simulink model "s_c_nbe_m32k"  (R2018a)
settings: Solver=VariableStepDiscrete  StartTime=0.0  StopTime=1000  RelTol=1e-3
undefined symbols (not defined in the file): fft_stages, n_taps, output_bits, pfb_coeff_gen_calc, xengbits
libraries: xbsIndex_r4 x23714, casper_library_misc x17, xps_library x4, casper_library_scopes x4, xbsReplacements_r4 x4
(part 45 of 171)

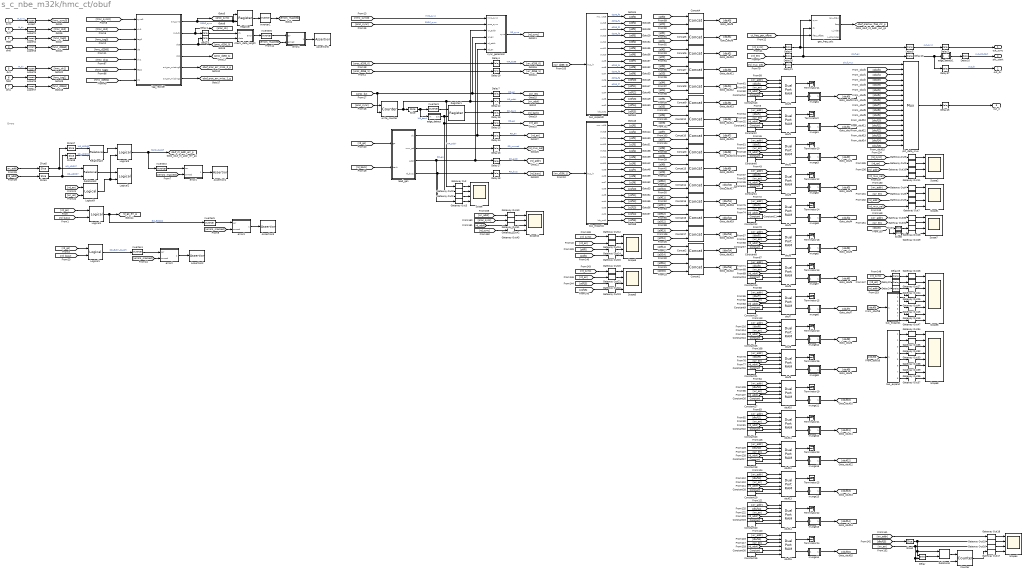
== system s_c_nbe_m32k/hmc_ct/obuf ==
  note: Errors
  sync : Inport
  dv0 : Inport  Port=2
  tag0 : Inport  Port=3
  din0 : Inport  Port=4
  dv1 : Inport  Port=5
  tag1 : Inport  Port=6
  din1 : Inport  Port=7
  Assert : xbsIndex_r4/Assert  assert_type=on  type_source=Explicitly  gui_display_data_type=Boolean  arith_type=Boolean  n_bits=16  bin_pt=14  preci_type=Single  exp_width=8  frac_width=24  assert_rate=on  rate_source=Explicitly  period=1  output_port=on  block_type=assert
  Assert1 : xbsIndex_r4/Assert  assert_type=on  type_source=Explicitly  gui_display_data_type=Boolean  arith_type=Boolean  n_bits=16  bin_pt=14  preci_type=Single  exp_width=8  frac_width=24  assert_rate=on  rate_source=Explicitly  period=1  output_port=on  block_type=assert
  Assert2 : xbsIndex_r4/Assert  assert_type=on  type_source=Explicitly  gui_display_data_type=Fixed-point  arith_type=Unsigned  n_bits=9  bin_pt=0  preci_type=Single  exp_width=8  frac_width=24  assert_rate=on  rate_source=Explicitly  period=1  output_port=on  block_type=assert
  Assert3 : xbsIndex_r4/Assert  assert_type=on  type_source=Explicitly  gui_display_data_type=Fixed-point  arith_type=Unsigned  n_bits=256  bin_pt=0  preci_type=Single  exp_width=8  frac_width=24  assert_rate=on  rate_source=Explicitly  period=1  output_port=on  block_type=assert
  Assert5 : xbsIndex_r4/Assert  assert_type=on  type_source=Explicitly  gui_display_data_type=Boolean  arith_type=Boolean  n_bits=16  bin_pt=14  preci_type=Single  exp_width=8  frac_width=24  assert_rate=on  rate_source=Explicitly  period=1  output_port=on  block_type=assert
  Assert6 : xbsIndex_r4/Assert  assert_type=on  type_source=Explicitly  gui_display_data_type=Fixed-point  arith_type=Unsigned  n_bits=9  bin_pt=0  preci_type=Single  exp_width=8  frac_width=24  assert_rate=on  rate_source=Explicitly  period=1  output_port=on  block_type=assert
  Assert7 : xbsIndex_r4/Assert  assert_type=on  type_source=Explicitly  gui_display_data_type=Fixed-point  arith_type=Unsigned  n_bits=256  bin_pt=0  preci_type=Single  exp_width=8  frac_width=24  assert_rate=on  rate_source=Explicitly  period=1  output_port=on  block_type=assert
  Assertion{1..3,5} (4 alike) : Assertion  Enabled=off
  Concat{1..10,12..17} (16 alike) : xbsIndex_r4/Concat  num_inputs=2  dbl_ovrd=off  block_type=concat
  Constant{1,3,5,7,9,11,13,15,17,19,22,24,26,28,30,42} (16 alike) : xbsIndex_r4/Constant  const=0  gui_display_data_type=Fixed-point  arith_type=Unsigned  n_bits=256  bin_pt=0  preci_type=Single  exp_width=8  frac_width=24  explicit_period=on  period=1  equ=P=C  opselect=C  inp2=PCIN>>17  opr=+  inp1=P  carry=CIN  dbl_ovrd=off  block_type=constant
  Constant{2,4,6,8,10,12,14,16,18,20..21,23,25,27,29,43} (16 alike) : xbsIndex_r4/Constant  const=0  gui_display_data_type=Boolean  arith_type=Boolean  n_bits=256  bin_pt=0  preci_type=Single  exp_width=8  frac_width=24  explicit_period=on  period=1  equ=P=C  opselect=C  inp2=PCIN>>17  opr=+  inp1=P  carry=CIN  dbl_ovrd=off  block_type=constant
  Counter : xbsIndex_r4/Counter  cnt_type=Free Running  cnt_to=Inf  operation=Up  start_count=0  cnt_by_val=1  arith_type=Unsigned  n_bits=8  bin_pt=0  load_pin=off  rst=on  en=on  explicit_period=on  period=1  use_behavioral_HDL=off  implementation=Fabric  dbl_ovrd=off  block_type=counter
  Delay : xbsIndex_r4/Delay  rst=off  infoeditControl=Selection of Reset will increase slice count due to use of real FFs and instead of SRLs  en=on  latency=1  reg_retiming=off  dbl_ovrd=off  block_type=delay
      settings: infoedit=Hardware notes: A delay line is a chain, each link of which is an SRL16 or SRL32 followed by a flip-flop.
  Delay1 : xbsIndex_r4/Delay  rst=off  infoeditControl=Selection of Reset will increase slice count due to use of real FFs and instead of SRLs  en=off  latency=1  reg_retiming=on  dbl_ovrd=off  block_type=delay
      settings: infoedit=Hardware notes: A delay line is a chain, each link of which is an SRL16 or SRL32 followed by a flip-flop.
  Delay{4,7,10,12..19} (11 alike) : xbsIndex_r4/Delay  rst=off  infoeditControl=Selection of Reset will increase slice count due to use of real FFs and instead of SRLs  en=off  latency=2  reg_retiming=on  dbl_ovrd=off  block_type=delay
      settings: infoedit=Hardware notes: A delay line is a chain, each link of which is an SRL16 or SRL32 followed by a flip-flop.
  Delay2 : xbsIndex_r4/Delay  rst=off  infoeditControl=Selection of Reset will increase slice count due to use of real FFs and instead of SRLs  en=off  latency=1  reg_retiming=on  dbl_ovrd=off  block_type=delay
      settings: infoedit=Hardware notes: A delay line is a chain, each link of which is an SRL16 or SRL32 followed by a flip-flop.
  Delay{6,20..24} (6 alike) : xbsIndex_r4/Delay  rst=off  infoeditControl=Selection of Reset will increase slice count due to use of real FFs and instead of SRLs  en=off  latency=pkt_buffer_latency  reg_retiming=on  dbl_ovrd=off  block_type=delay
      settings: infoedit=Hardware notes: A delay line is a chain, each link of which is an SRL16 or SRL32 followed by a flip-flop.
  Delay3 : xbsIndex_r4/Delay  rst=off  infoeditControl=Selection of Reset will increase slice count due to use of real FFs and instead of SRLs  en=off  latency=3  reg_retiming=on  dbl_ovrd=off  block_type=delay
      settings: infoedit=Hardware notes: A delay line is a chain, each link of which is an SRL16 or SRL32 followed by a flip-flop.
  Delay37 : xbsIndex_r4/Delay  rst=off  infoeditControl=Selection of Reset will increase slice count due to use of real FFs and instead of SRLs  en=off  latency=3  reg_retiming=on  dbl_ovrd=off  block_type=delay
      settings: infoedit=Hardware notes: A delay line is a chain, each link of which is an SRL16 or SRL32 followed by a flip-flop.
  Delay43 : xbsIndex_r4/Delay  rst=off  infoeditControl=Selection of Reset will increase slice count due to use of real FFs and instead of SRLs  en=off  latency=omux_latency  reg_retiming=on  dbl_ovrd=off  block_type=delay
      settings: infoedit=Hardware notes: A delay line is a chain, each link of which is an SRL16 or SRL32 followed by a flip-flop.
  Delay45 : xbsIndex_r4/Delay  rst=off  infoeditControl=Selection of Reset will increase slice count due to use of real FFs and instead of SRLs  en=off  latency=3  reg_retiming=on  dbl_ovrd=off  block_type=delay
      settings: infoedit=Hardware notes: A delay line is a chain, each link of which is an SRL16 or SRL32 followed by a flip-flop.
  Delay5 : xbsIndex_r4/Delay  rst=off  infoeditControl=Selection of Reset will increase slice count due to use of real FFs and instead of SRLs  en=off  latency=omux_latency  reg_retiming=on  dbl_ovrd=off  block_type=delay
      settings: infoedit=Hardware notes: A delay line is a chain, each link of which is an SRL16 or SRL32 followed by a flip-flop.
  Gateway Out{,1..47} (48 alike) : xbsIndex_r4/Gateway Out  inherit_from_input=off  hdl_port=off  rows=1  columns=1  UseAsDAC=off  DACChannel='1'  interface=None  automatic_assignment=on  address_offset=hex2dec('00')  intf_name=''  intf_description=''  timing_constraint=None  locs_specified=off  LOCs={}  io_standard={}  block_type=gatewayout
  Inverter{1..6} (6 alike) : xbsIndex_r4/Inverter  en=off  latency=0  dbl_ovrd=off  block_type=inv
  Logical1 : xbsIndex_r4/Logical  logical_function=AND  inputs=2  en=off  latency=1  precision=Full  arith_type=Unsigned  n_bits=16  bin_pt=0  align_bp=on  dbl_ovrd=off  block_type=logical
  Logical2 : xbsIndex_r4/Logical  logical_function=AND  inputs=2  en=off  latency=0  precision=Full  arith_type=Unsigned  n_bits=16  bin_pt=0  align_bp=on  dbl_ovrd=off  block_type=logical
  Logical3 : xbsIndex_r4/Logical  logical_function=AND  inputs=2  en=off  latency=0  precision=Full  arith_type=Unsigned  n_bits=16  bin_pt=0  align_bp=on  dbl_ovrd=off  block_type=logical
  Logical4 : xbsIndex_r4/Logical  logical_function=AND  inputs=2  en=off  latency=1  precision=Full  arith_type=Unsigned  n_bits=16  bin_pt=0  align_bp=on  dbl_ovrd=off  block_type=logical
  Logical9 : xbsIndex_r4/Logical  logical_function=AND  inputs=2  en=off  latency=0  precision=Full  arith_type=Unsigned  n_bits=16  bin_pt=0  align_bp=on  dbl_ovrd=off  block_type=logical
  Register : xbsIndex_r4/Register  init=0  rst=off  en=on  dbl_ovrd=off  block_type=register
  Register1 : xbsIndex_r4/Register  init=0  rst=off  en=on  dbl_ovrd=off  block_type=register
  Relational : xbsIndex_r4/Relational  mode=a!=b  op_type=Bool  en=off  latency=0  dbl_ovrd=off  block_type=relational
  Relational2 : xbsIndex_r4/Relational  mode=a=b  op_type=Bool  en=off  latency=0  dbl_ovrd=off  block_type=relational
  Relational3 : xbsIndex_r4/Relational  mode=a=b  op_type=Bool  en=off  latency=0  dbl_ovrd=off  block_type=relational
  Scope{,1..5,7,10} (8 alike) : Scope  NumInputPorts=4
  Scope6 : Scope  NumInputPorts=8
  Scope8 : Scope  NumInputPorts=8
  Slice : xbsIndex_r4/Slice  nbits=1  boolean_output=on  mode=Upper Bit Location + Width  bit1=0  base1=MSB of Input  bit0=0  base0=LSB of Input  dbl_ovrd=off  block_type=slice
  Slice1 : xbsIndex_r4/Slice  nbits=1  boolean_output=off  mode=Two Bit Locations  bit1=0  base1=MSB of Input  bit0=0  base0=LSB of Input  dbl_ovrd=off  block_type=slice
  Slice17 : xbsIndex_r4/Slice  nbits=1  boolean_output=off  mode=Two Bit Locations  bit1=0  base1=MSB of Input  bit0=5  base0=LSB of Input  dbl_ovrd=off  block_type=slice
  Slice18 : xbsIndex_r4/Slice  nbits=1  boolean_output=off  mode=Two Bit Locations  bit1=0  base1=MSB of Input  bit0=5  base0=LSB of Input  dbl_ovrd=off  block_type=slice
  Slice2 : xbsIndex_r4/Slice  nbits=16  boolean_output=off  mode=Lower Bit Location + Width  bit1=0  base1=MSB of Input  bit0=0  base0=LSB of Input  dbl_ovrd=off  block_type=slice
  Slice5 : xbsIndex_r4/Slice  nbits=1  boolean_output=off  mode=Two Bit Locations  bit1=0  base1=MSB of Input  bit0=3  base0=LSB of Input  dbl_ovrd=off  block_type=slice
  Slice7 : xbsIndex_r4/Slice  nbits=16  boolean_output=off  mode=Lower Bit Location + Width  bit1=0  base1=MSB of Input  bit0=16  base0=LSB of Input  dbl_ovrd=off  block_type=slice
  Slice8 : xbsIndex_r4/Slice  nbits=16  boolean_output=off  mode=Lower Bit Location + Width  bit1=0  base1=MSB of Input  bit0=16  base0=LSB of Input  dbl_ovrd=off  block_type=slice
  Terminator{2,10..15,18..26} (16 alike) : Terminator
  bus_expand : Subsystem  mask(bus_expand){mode=divisions of equal size, outputNum=8, outputWidth=16, outputBinaryPt=0, outputArithmeticType=0, show_format=off, outputToWorkspace=off, variablePrefix=out, outputToModelAsWell=on}
      mask prompts: outputNum "Number of outputs:"; outputWidth "Output width:"; outputBinaryPt "Output binary point position:"; outputArithmeticType "Output arithmetic type (ufix=0, fix=1, bool=2):"; show_format "Print format string?"; outputToWorkspace "Output to workspace?"; variablePrefix "Variable name prefix:"; outputToModelAsWell "Output to model as well?"
      mask help:
      | Expands a 'bus' made using a bus_create or Xilinx
      | concat block.
      | The input will be divided into the specified number
      | of outputs with the specified arithmetic types.
      | Divisions are made from most significant bit.
      mask init: same as s_c_nbe_m32k/bus_expand1
      settings: AttributesFormatString=8 outputs
      mask TypeOptions mode: divisions of equal size | divisions of arbitrary size
      mask Callback mode: bus_expand_callback();
      mask Callback outputWidth: bus_expand_callback();
      mask Callback outputToWorkspace: bus_expand_callback();
  bus_expand1 : Subsystem  mask(bus_expand){mode=divisions of equal size, outputNum=8, outputWidth=16, outputBinaryPt=0, outputArithmeticType=0, show_format=off, outputToWorkspace=off, variablePrefix=out, outputToModelAsWell=on}
      mask prompts: outputNum "Number of outputs:"; outputWidth "Output width:"; outputBinaryPt "Output binary point position:"; outputArithmeticType "Output arithmetic type (ufix=0, fix=1, bool=2):"; show_format "Print format string?"; outputToWorkspace "Output to workspace?"; variablePrefix "Variable name prefix:"; outputToModelAsWell "Output to model as well?"
      mask help:
      | Expands a 'bus' made using a bus_create or Xilinx
      | concat block.
      | The input will be divided into the specified number
      | of outputs with the specified arithmetic types.
      | Divisions are made from most significant bit.
      mask init: same as s_c_nbe_m32k/bus_expand1
      settings: AttributesFormatString=8 outputs
      mask TypeOptions mode: divisions of equal size | divisions of arbitrary size
      mask Callback mode: bus_expand_callback();
      mask Callback outputWidth: bus_expand_callback();
      mask Callback outputToWorkspace: bus_expand_callback();
  bus_expand2 : Subsystem  mask(bus_expand){mode=divisions of equal size, outputNum=16, outputWidth=16, outputBinaryPt=0, outputArithmeticType=0, show_format=off, outputToWorkspace=off, variablePrefix=out, outputToModelAsWell=on}
      mask prompts: outputNum "Number of outputs:"; outputWidth "Output width:"; outputBinaryPt "Output binary point position:"; outputArithmeticType "Output arithmetic type (ufix=0, fix=1, bool=2):"; show_format "Print format string?"; outputToWorkspace "Output to workspace?"; variablePrefix "Variable name prefix:"; outputToModelAsWell "Output to model as well?"
      mask help:
      | Expands a 'bus' made using a bus_create or Xilinx
      | concat block.
      | The input will be divided into the specified number
      | of outputs with the specified arithmetic types.
      | Divisions are made from most significant bit.
      mask init: same as s_c_nbe_m32k/bus_expand1
      settings: AttributesFormatString=16 outputs
      mask TypeOptions mode: divisions of equal size | divisions of arbitrary size
      mask Callback mode: bus_expand_callback();
      mask Callback outputWidth: bus_expand_callback();
      mask Callback outputToWorkspace: bus_expand_callback();
  bus_expand4 : Subsystem  mask(bus_expand){mode=divisions of equal size, outputNum=16, outputWidth=16, outputBinaryPt=0, outputArithmeticType=0, show_format=off, outputToWorkspace=off, variablePrefix=out, outputToModelAsWell=on}
      mask prompts: outputNum "Number of outputs:"; outputWidth "Output width:"; outputBinaryPt "Output binary point position:"; outputArithmeticType "Output arithmetic type (ufix=0, fix=1, bool=2):"; show_format "Print format string?"; outputToWorkspace "Output to workspace?"; variablePrefix "Variable name prefix:"; outputToModelAsWell "Output to model as well?"
      mask help:
      | Expands a 'bus' made using a bus_create or Xilinx
      | concat block.
      | The input will be divided into the specified number
      | of outputs with the specified arithmetic types.
      | Divisions are made from most significant bit.
      mask init: same as s_c_nbe_m32k/bus_expand1
      settings: AttributesFormatString=16 outputs
      mask TypeOptions mode: divisions of equal size | divisions of arbitrary size
      mask Callback mode: bus_expand_callback();
      mask Callback outputWidth: bus_expand_callback();
      mask Callback outputToWorkspace: bus_expand_callback();
  check_data_length : Subsystem
  edge_detect : Subsystem  mask(edge_detect){edge=Both, polarity=Active High, x_in=[0 0.08 0.08 0.16 0.16 0.24 0.24 0.32 0.32 0.4], y_in=[-1 -1  1  1  1  1  1  1  1  1], x_out=[0.6 0.68 0.68 0.76 0.76 0.84 0.84 0.92 0.92 1], y_out=[-1 -1  1  1 -1 -1 -1 -1 -1 -1]}
      mask prompts: edge "Edge Type"; polarity "Output Polarity"; x_in "Input X Positions"; y_in "Input Y Positions"; x_out "Output X Positions"; y_out "Output Y Positions"
      mask help: Output is active for one-cycle after each edge of the specified type (i.e. rising, falling or both).
      mask init: same as s_c_nbe_m32k/edge_detect1
      settings: AttributesFormatString=|
      | both edges
      | active high
      mask Help: Output is active for one-cycle after each edge of the specified type (i.e. rising, falling, or both).  Latency is zero.
      mask TypeOptions edge: Rising | Falling | Both
      mask TypeOptions polarity: Active High | Active Low
      mask Display:
      | plot(x_in_num,0.5+y_in_num*0.2);
      | plot(x_out_num,0.5+y_out_num*0.2);
  edge_detect1 : Subsystem  mask(edge_detect){edge=Rising, polarity=Active High, x_in=[0 0.08 0.08 0.16 0.16 0.24 0.24 0.32 0.32 0.4], y_in=[-1 -1  1  1  1  1  1  1  1  1], x_out=[0.6 0.68 0.68 0.76 0.76 0.84 0.84 0.92 0.92 1], y_out=[-1 -1  1  1 -1 -1 -1 -1 -1 -1]}
      mask prompts: edge "Edge Type"; polarity "Output Polarity"; x_in "Input X Positions"; y_in "Input Y Positions"; x_out "Output X Positions"; y_out "Output Y Positions"
      mask help: Output is active for one-cycle after each edge of the specified type (i.e. rising, falling or both).
      mask init: same as s_c_nbe_m32k/edge_detect1
      settings: AttributesFormatString=|
      | rising edges
      | active high
      mask Help: Output is active for one-cycle after each edge of the specified type (i.e. rising, falling, or both).  Latency is zero.
      mask TypeOptions edge: Rising | Falling | Both
      mask TypeOptions polarity: Active High | Active Low
      mask Display:
      | plot(x_in_num,0.5+y_in_num*0.2);
      | plot(x_out_num,0.5+y_out_num*0.2);
  error1 : Subsystem
  error2 : Subsystem
  error3 : Subsystem
  error4 : Subsystem
  gen_freq_calc : Subsystem  mask{pkt_len_bits=5, lat=3}
      mask prompts: pkt_len_bits "Packet length bits"; lat "Latency"
      mask init:
      | display_string = sprintf('latency=%i', 7 * lat);
      | set_param(gcb, 'AttributesFormatString', display_string);
      settings: AttributesFormatString=latency=21
  munge1 : Subsystem  mask(munge){divisions=8, div_size=[32 32 32 32 32 32 32 32], order=[7 6 5 4 3 2 1 0], arith_type_out=Unsigned, bin_pt_out=0}
      mask prompts: divisions "Number of divisions"; div_size "Division size (bits)"; order "Division packing order"; arith_type_out "Output arithmetic type"; bin_pt_out "Output binary point"
      mask help: Splits an input bus into the specified number of divisions and then recombines them in the order specified (most significant division = 0,least = number divisions-1)
      mask init:
      | munge_init(gcb, ...
      |     'divisions', divisions, ...
      |     'div_size', div_size, ...
      |     'order', order, ...
      |     'arith_type_out', arith_type_out, ...
      |     'bin_pt_out', bin_pt_out);
      settings: AttributesFormatString=|
      | split:[32 32 32 32 32 32 32 32]
      | join:[7 6 5 4 3 2 1 0]
      | Unsigned [256,0]
      mask TypeOptions arith_type_out: Unsigned | Signed  (2's comp) | Floating-point
  munge10 : Subsystem  mask(munge){divisions=8, div_size=[32 32 32 32 32 32 32 32], order=[7 6 5 4 3 2 1 0], arith_type_out=Unsigned, bin_pt_out=0}
      mask prompts: divisions "Number of divisions"; div_size "Division size (bits)"; order "Division packing order"; arith_type_out "Output arithmetic type"; bin_pt_out "Output binary point"
      mask help: Splits an input bus into the specified number of divisions and then recombines them in the order specified (most significant division = 0,least = number divisions-1)
      mask init:
      | munge_init(gcb, ...
      |     'divisions', divisions, ...
      |     'div_size', div_size, ...
      |     'order', order, ...
      |     'arith_type_out', arith_type_out, ...
      |     'bin_pt_out', bin_pt_out);
      settings: AttributesFormatString=|
      | split:[32 32 32 32 32 32 32 32]
      | join:[7 6 5 4 3 2 1 0]
      | Unsigned [256,0]
      mask TypeOptions arith_type_out: Unsigned | Signed  (2's comp) | Floating-point
  munge11 : Subsystem  mask(munge){divisions=8, div_size=[32 32 32 32 32 32 32 32], order=[7 6 5 4 3 2 1 0], arith_type_out=Unsigned, bin_pt_out=0}
      mask prompts: divisions "Number of divisions"; div_size "Division size (bits)"; order "Division packing order"; arith_type_out "Output arithmetic type"; bin_pt_out "Output binary point"
      mask help: Splits an input bus into the specified number of divisions and then recombines them in the order specified (most significant division = 0,least = number divisions-1)
      mask init:
      | munge_init(gcb, ...
      |     'divisions', divisions, ...
      |     'div_size', div_size, ...
      |     'order', order, ...
      |     'arith_type_out', arith_type_out, ...
      |     'bin_pt_out', bin_pt_out);
      settings: AttributesFormatString=|
      | split:[32 32 32 32 32 32 32 32]
      | join:[7 6 5 4 3 2 1 0]
      | Unsigned [256,0]
      mask TypeOptions arith_type_out: Unsigned | Signed  (2's comp) | Floating-point
  munge12 : Subsystem  mask(munge){divisions=8, div_size=[32 32 32 32 32 32 32 32], order=[7 6 5 4 3 2 1 0], arith_type_out=Unsigned, bin_pt_out=0}
      mask prompts: divisions "Number of divisions"; div_size "Division size (bits)"; order "Division packing order"; arith_type_out "Output arithmetic type"; bin_pt_out "Output binary point"
      mask help: Splits an input bus into the specified number of divisions and then recombines them in the order specified (most significant division = 0,least = number divisions-1)
      mask init:
      | munge_init(gcb, ...
      |     'divisions', divisions, ...
      |     'div_size', div_size, ...
      |     'order', order, ...
      |     'arith_type_out', arith_type_out, ...
      |     'bin_pt_out', bin_pt_out);
      settings: AttributesFormatString=|
      | split:[32 32 32 32 32 32 32 32]
      | join:[7 6 5 4 3 2 1 0]
      | Unsigned [256,0]
      mask TypeOptions arith_type_out: Unsigned | Signed  (2's comp) | Floating-point
  munge13 : Subsystem  mask(munge){divisions=8, div_size=[32 32 32 32 32 32 32 32], order=[7 6 5 4 3 2 1 0], arith_type_out=Unsigned, bin_pt_out=0}
      mask prompts: divisions "Number of divisions"; div_size "Division size (bits)"; order "Division packing order"; arith_type_out "Output arithmetic type"; bin_pt_out "Output binary point"
      mask help: Splits an input bus into the specified number of divisions and then recombines them in the order specified (most significant division = 0,least = number divisions-1)
      mask init:
      | munge_init(gcb, ...
      |     'divisions', divisions, ...
      |     'div_size', div_size, ...
      |     'order', order, ...
      |     'arith_type_out', arith_type_out, ...
      |     'bin_pt_out', bin_pt_out);
      settings: AttributesFormatString=|
      | split:[32 32 32 32 32 32 32 32]
      | join:[7 6 5 4 3 2 1 0]
      | Unsigned [256,0]
      mask TypeOptions arith_type_out: Unsigned | Signed  (2's comp) | Floating-point
  munge14 : Subsystem  mask(munge){divisions=8, div_size=[32 32 32 32 32 32 32 32], order=[7 6 5 4 3 2 1 0], arith_type_out=Unsigned, bin_pt_out=0}
      mask prompts: divisions "Number of divisions"; div_size "Division size (bits)"; order "Division packing order"; arith_type_out "Output arithmetic type"; bin_pt_out "Output binary point"
      mask help: Splits an input bus into the specified number of divisions and then recombines them in the order specified (most significant division = 0,least = number divisions-1)
      mask init:
      | munge_init(gcb, ...
      |     'divisions', divisions, ...
      |     'div_size', div_size, ...
      |     'order', order, ...
      |     'arith_type_out', arith_type_out, ...
      |     'bin_pt_out', bin_pt_out);
      settings: AttributesFormatString=|
      | split:[32 32 32 32 32 32 32 32]
      | join:[7 6 5 4 3 2 1 0]
      | Unsigned [256,0]
      mask TypeOptions arith_type_out: Unsigned | Signed  (2's comp) | Floating-point
  munge15 : Subsystem  mask(munge){divisions=8, div_size=[32 32 32 32 32 32 32 32], order=[7 6 5 4 3 2 1 0], arith_type_out=Unsigned, bin_pt_out=0}
      mask prompts: divisions "Number of divisions"; div_size "Division size (bits)"; order "Division packing order"; arith_type_out "Output arithmetic type"; bin_pt_out "Output binary point"
      mask help: Splits an input bus into the specified number of divisions and then recombines them in the order specified (most significant division = 0,least = number divisions-1)
      mask init:
      | munge_init(gcb, ...
      |     'divisions', divisions, ...
      |     'div_size', div_size, ...
      |     'order', order, ...
      |     'arith_type_out', arith_type_out, ...
      |     'bin_pt_out', bin_pt_out);
      settings: AttributesFormatString=|
      | split:[32 32 32 32 32 32 32 32]
      | join:[7 6 5 4 3 2 1 0]
      | Unsigned [256,0]
      mask TypeOptions arith_type_out: Unsigned | Signed  (2's comp) | Floating-point
  munge16 : Subsystem  mask(munge){divisions=8, div_size=[32 32 32 32 32 32 32 32], order=[7 6 5 4 3 2 1 0], arith_type_out=Unsigned, bin_pt_out=0}
      mask prompts: divisions "Number of divisions"; div_size "Division size (bits)"; order "Division packing order"; arith_type_out "Output arithmetic type"; bin_pt_out "Output binary point"
      mask help: Splits an input bus into the specified number of divisions and then recombines them in the order specified (most significant division = 0,least = number divisions-1)
      mask init:
      | munge_init(gcb, ...
      |     'divisions', divisions, ...
      |     'div_size', div_size, ...
      |     'order', order, ...
      |     'arith_type_out', arith_type_out, ...
      |     'bin_pt_out', bin_pt_out);
      settings: AttributesFormatString=|
      | split:[32 32 32 32 32 32 32 32]
      | join:[7 6 5 4 3 2 1 0]
      | Unsigned [256,0]
      mask TypeOptions arith_type_out: Unsigned | Signed  (2's comp) | Floating-point
  munge2 : Subsystem  mask(munge){divisions=8, div_size=[32 32 32 32 32 32 32 32], order=[7 6 5 4 3 2 1 0], arith_type_out=Unsigned, bin_pt_out=0}
      mask prompts: divisions "Number of divisions"; div_size "Division size (bits)"; order "Division packing order"; arith_type_out "Output arithmetic type"; bin_pt_out "Output binary point"
      mask help: Splits an input bus into the specified number of divisions and then recombines them in the order specified (most significant division = 0,least = number divisions-1)
      mask init:
      | munge_init(gcb, ...
      |     'divisions', divisions, ...
      |     'div_size', div_size, ...
      |     'order', order, ...
      |     'arith_type_out', arith_type_out, ...
      |     'bin_pt_out', bin_pt_out);
      settings: AttributesFormatString=|
      | split:[32 32 32 32 32 32 32 32]
      | join:[7 6 5 4 3 2 1 0]
      | Unsigned [256,0]
      mask TypeOptions arith_type_out: Unsigned | Signed  (2's comp) | Floating-point
  munge3 : Subsystem  mask(munge){divisions=8, div_size=[32 32 32 32 32 32 32 32], order=[7 6 5 4 3 2 1 0], arith_type_out=Unsigned, bin_pt_out=0}
      mask prompts: divisions "Number of divisions"; div_size "Division size (bits)"; order "Division packing order"; arith_type_out "Output arithmetic type"; bin_pt_out "Output binary point"
      mask help: Splits an input bus into the specified number of divisions and then recombines them in the order specified (most significant division = 0,least = number divisions-1)
      mask init:
      | munge_init(gcb, ...
      |     'divisions', divisions, ...
      |     'div_size', div_size, ...
      |     'order', order, ...
      |     'arith_type_out', arith_type_out, ...
      |     'bin_pt_out', bin_pt_out);
      settings: AttributesFormatString=|
      | split:[32 32 32 32 32 32 32 32]
      | join:[7 6 5 4 3 2 1 0]
      | Unsigned [256,0]
      mask TypeOptions arith_type_out: Unsigned | Signed  (2's comp) | Floating-point
  munge4 : Subsystem  mask(munge){divisions=8, div_size=[32 32 32 32 32 32 32 32], order=[7 6 5 4 3 2 1 0], arith_type_out=Unsigned, bin_pt_out=0}
      mask prompts: divisions "Number of divisions"; div_size "Division size (bits)"; order "Division packing order"; arith_type_out "Output arithmetic type"; bin_pt_out "Output binary point"
      mask help: Splits an input bus into the specified number of divisions and then recombines them in the order specified (most significant division = 0,least = number divisions-1)
      mask init:
      | munge_init(gcb, ...
      |     'divisions', divisions, ...
      |     'div_size', div_size, ...
      |     'order', order, ...
      |     'arith_type_out', arith_type_out, ...
      |     'bin_pt_out', bin_pt_out);
      settings: AttributesFormatString=|
      | split:[32 32 32 32 32 32 32 32]
      | join:[7 6 5 4 3 2 1 0]
      | Unsigned [256,0]
      mask TypeOptions arith_type_out: Unsigned | Signed  (2's comp) | Floating-point
  munge5 : Subsystem  mask(munge){divisions=8, div_size=[32 32 32 32 32 32 32 32], order=[7 6 5 4 3 2 1 0], arith_type_out=Unsigned, bin_pt_out=0}
      mask prompts: divisions "Number of divisions"; div_size "Division size (bits)"; order "Division packing order"; arith_type_out "Output arithmetic type"; bin_pt_out "Output binary point"
      mask help: Splits an input bus into the specified number of divisions and then recombines them in the order specified (most significant division = 0,least = number divisions-1)
      mask init:
      | munge_init(gcb, ...
      |     'divisions', divisions, ...
      |     'div_size', div_size, ...
      |     'order', order, ...
      |     'arith_type_out', arith_type_out, ...
      |     'bin_pt_out', bin_pt_out);
      settings: AttributesFormatString=|
      | split:[32 32 32 32 32 32 32 32]
      | join:[7 6 5 4 3 2 1 0]
      | Unsigned [256,0]
      mask TypeOptions arith_type_out: Unsigned | Signed  (2's comp) | Floating-point
  munge6 : Subsystem  mask(munge){divisions=8, div_size=[32 32 32 32 32 32 32 32], order=[7 6 5 4 3 2 1 0], arith_type_out=Unsigned, bin_pt_out=0}
      mask prompts: divisions "Number of divisions"; div_size "Division size (bits)"; order "Division packing order"; arith_type_out "Output arithmetic type"; bin_pt_out "Output binary point"
      mask help: Splits an input bus into the specified number of divisions and then recombines them in the order specified (most significant division = 0,least = number divisions-1)
      mask init:
      | munge_init(gcb, ...
      |     'divisions', divisions, ...
      |     'div_size', div_size, ...
      |     'order', order, ...
      |     'arith_type_out', arith_type_out, ...
      |     'bin_pt_out', bin_pt_out);
      settings: AttributesFormatString=|
      | split:[32 32 32 32 32 32 32 32]
      | join:[7 6 5 4 3 2 1 0]
      | Unsigned [256,0]
      mask TypeOptions arith_type_out: Unsigned | Signed  (2's comp) | Floating-point
  munge7 : Subsystem  mask(munge){divisions=8, div_size=[32 32 32 32 32 32 32 32], order=[7 6 5 4 3 2 1 0], arith_type_out=Unsigned, bin_pt_out=0}
      mask prompts: divisions "Number of divisions"; div_size "Division size (bits)"; order "Division packing order"; arith_type_out "Output arithmetic type"; bin_pt_out "Output binary point"
      mask help: Splits an input bus into the specified number of divisions and then recombines them in the order specified (most significant division = 0,least = number divisions-1)
      mask init:
      | munge_init(gcb, ...
      |     'divisions', divisions, ...
      |     'div_size', div_size, ...
      |     'order', order, ...
      |     'arith_type_out', arith_type_out, ...
      |     'bin_pt_out', bin_pt_out);
      settings: AttributesFormatString=|
      | split:[32 32 32 32 32 32 32 32]
      | join:[7 6 5 4 3 2 1 0]
      | Unsigned [256,0]
      mask TypeOptions arith_type_out: Unsigned | Signed  (2's comp) | Floating-point
  munge8 : Subsystem  mask(munge){divisions=8, div_size=[32 32 32 32 32 32 32 32], order=[7 6 5 4 3 2 1 0], arith_type_out=Unsigned, bin_pt_out=0}
      mask prompts: divisions "Number of divisions"; div_size "Division size (bits)"; order "Division packing order"; arith_type_out "Output arithmetic type"; bin_pt_out "Output binary point"
      mask help: Splits an input bus into the specified number of divisions and then recombines them in the order specified (most significant division = 0,least = number divisions-1)
      mask init:
      | munge_init(gcb, ...
      |     'divisions', divisions, ...
      |     'div_size', div_size, ...
      |     'order', order, ...
      |     'arith_type_out', arith_type_out, ...
      |     'bin_pt_out', bin_pt_out);
      settings: AttributesFormatString=|
      | split:[32 32 32 32 32 32 32 32]
      | join:[7 6 5 4 3 2 1 0]
      | Unsigned [256,0]
      mask TypeOptions arith_type_out: Unsigned | Signed  (2's comp) | Floating-point
  munge9 : Subsystem  mask(munge){divisions=8, div_size=[32 32 32 32 32 32 32 32], order=[7 6 5 4 3 2 1 0], arith_type_out=Unsigned, bin_pt_out=0}
      mask prompts: divisions "Number of divisions"; div_size "Division size (bits)"; order "Division packing order"; arith_type_out "Output arithmetic type"; bin_pt_out "Output binary point"
      mask help: Splits an input bus into the specified number of divisions and then recombines them in the order specified (most significant division = 0,least = number divisions-1)
      mask init:
      | munge_init(gcb, ...
      |     'divisions', divisions, ...
      |     'div_size', div_size, ...
      |     'order', order, ...
      |     'arith_type_out', arith_type_out, ...
      |     'bin_pt_out', bin_pt_out);
      settings: AttributesFormatString=|
      | split:[32 32 32 32 32 32 32 32]
      | join:[7 6 5 4 3 2 1 0]
      | Unsigned [256,0]
      mask TypeOptions arith_type_out: Unsigned | Signed  (2's comp) | Floating-point
  obuf{0..15} (16 alike) : xbsIndex_r4/Dual Port RAM  depth=2^(output_len_bits + 1)  initVector=ones(1, 2^(output_len_bits + 1))  distributed_mem=Block RAM  init_a=0  init_b=0  rst_a=off  rst_b=off  en_a=off  en_b=off  latency=pkt_buffer_latency  write_mode_A=Read Before Write  write_mode_B=Read Before Write  optimize=Area  dbl_ovrd=off  block_type=dpram
  pkt_data_mux : xbsIndex_r4/Mux  inputs=16  en=off  latency=omux_latency  precision=Full  arith_type=Unsigned  n_bits=16  bin_pt=14  quantization=Truncate  overflow=Wrap  dbl_ovrd=off  block_type=mux
  read_gen : Subsystem
  sync_generator : Subsystem
  tag_reorder : Subsystem
  write_counter : xbsIndex_r4/Counter  cnt_type=Free Running  cnt_to=Inf  operation=Up  start_count=0  cnt_by_val=1  arith_type=Unsigned  n_bits=9  bin_pt=0  load_pin=off  rst=on  en=on  explicit_period=on  period=1  use_behavioral_HDL=off  implementation=Fabric  dbl_ovrd=off  block_type=counter
  out_sync : Outport
  out_dv : Outport  Port=2
  out_d : Outport  Port=3
  pkt_start : Outport  Port=4
  tag scope: obuf_ct_addr_err_g=global, obuf_premux_freq_ctr_g=global, obuf_proc_err_miss_0_g=global, obuf_proc_err_miss_1_g=global, rd_go_err_g=global
  wires:
  dv0/1 -> Assert1/1  "IN_dv"
  tag0/1 -> Assert2/1
  sync/1 -> Assert/1  "IN_sync"
  [rd_en] -> Logical9/1
  [wr_en] -> Logical9/2
  Logical9/1 -> Logical3/2, Logical2/2
  [rd_go] -> Logical4/1
  [rd_busy] -> Logical4/2
  Logical4/1 -> Inverter5/1, [rd_go_err_g]  "GO_ERROR"
  din0/1 -> Assert3/1
  [wr_addr] -> Slice5/1
  [rd_addr] -> Slice1/1
  Slice5/1 -> Slice17/1, Relational2/1  "WR_ADDR7"
  Slice1/1 -> Slice18/1, Relational2/2  "RD_ADDR7"
  Relational2/1 -> Logical2/1
  Logical3/1 -> Inverter2/1, [obuf_ct_addr_err_g]  "BANK_CLASH"
  Slice18/1 -> Relational3/2  "RD_ADDR2"
  Slice17/1 -> Relational3/1  "WR_ADDR2"
  Relational3/1 -> Logical3/1
  [hmc_d2560] -> tag_reorder/4(d0)
  [hmc_tag0] -> tag_reorder/3(tag0)
  [hmc_dv0] -> tag_reorder/2(dv0)
  [hmc_sync0] -> tag_reorder/1(sync0)
  check_data_length/1(error) -> Inverter6/1
  tag_reorder/3(do0) -> [proc_d256_0], Delay2/1
  tag_reorder/2(out_dv) -> [proc_dv], Delay1/1
  Inverter6/1 -> error4/1(err)
  error4/1(err_out) -> Assertion5/1
  tag_reorder/1(out_sync) -> [proc_sync], Register/2, Register/1  "PROC_sync"
  Register/1 -> Inverter1/1
  Inverter1/1 -> [errors_masked]
  [errors_masked] -> error4/2(armed)
  Delay1/1 -> check_data_length/1(dv)
  Delay2/1 -> check_data_length/2(data)
  [rd_go] -> Logical1/1
  [rd_busy] -> Logical1/2
  Logical1/1 -> Inverter4/1  "RD_BUSY_CLASH"
  Inverter4/1 -> error2/1(err)
  error2/1(err_out) -> Assertion2/1
  [errors_masked] -> error2/2(armed)
  [dbuf0] -> obuf0/2
  [wr_addr] -> obuf0/1
  [wr_en] -> obuf0/3
  [rd_addr] -> obuf0/4
  Constant42/1 -> obuf0/5
  Constant43/1 -> obuf0/6
  obuf0/2 -> munge4/1(din)
  obuf0/1 -> Terminator11/1
  [rd_mux_sel] -> Delay21/1
  [obuf4] -> pkt_data_mux/6
  [obuf6] -> pkt_data_mux/8
  [obuf5] -> pkt_data_mux/7
  [obuf7] -> pkt_data_mux/9
  [obuf3] -> pkt_data_mux/5
  [obuf2] -> pkt_data_mux/4
  [obuf0] -> pkt_data_mux/2
  [obuf1] -> pkt_data_mux/3
  [rd_en] -> Delay20/1
  Delay45/1 -> out_d/1
  Delay37/1 -> out_dv/1  "out_dv"
  pkt_data_mux/1 -> Delay45/1
  Delay21/1 -> pkt_data_mux/1  "obuf_mux"
  Delay20/1 -> Delay43/1, gen_freq_calc/2(dv)  "obuf_en"
  Delay5/1 -> Delay3/1  "out_sync"
  edge_detect1/1(out) -> Delay10/1
  Delay43/1 -> Delay37/1, edge_detect1/1(in)
  Delay10/1 -> pkt_start/1  "out_pkt_start"
  Delay6/1 -> Delay5/1, gen_freq_calc/1(sync)
  Assert/1 -> [hmc_sync0]
  Assert1/1 -> [hmc_dv0]
  Assert2/1 -> [hmc_tag0]
  Assert3/1 -> [hmc_d2560]
  Inverter2/1 -> error1/1(err)
  error1/1(err_out) -> Assertion1/1
  [errors_masked] -> error1/2(armed)
  Inverter5/1 -> error3/1(err)
  error3/1(err_out) -> Assertion3/1
  [errors_masked] -> error3/2(armed)
  Delay3/1 -> out_sync/1
  gen_freq_calc/2(freq) -> [obuf_premux_freq_ctr_g]
  [proc_sync] -> write_counter/1
  [proc_dv] -> sync_generator/4(wr_en), Delay7/1, write_counter/2
  write_counter/1 -> Gateway Out/1, sync_generator/3(wr_addr), Delay12/1, Slice/1  "WR_addr"
  Slice/1 -> Inverter3/1, edge_detect/1(in)  "WR_bank"
  Inverter3/1 -> Register1/1
  edge_detect/1(out) -> Delay15/1, Gateway Out1/1, Register1/2  "RD_go"
  Register1/1 -> Delay16/1
  read_gen/2(mux_sel) -> Delay13/1
  read_gen/1(dv) -> Delay14/1, sync_generator/6(rd_en)
  read_gen/3(addr) -> Gateway Out3/1, Delay17/1, sync_generator/5(rd_addr)
  read_gen/4(rd_busy) -> Gateway Out2/1, Delay18/1
  [rd_bank] -> read_gen/2(bank)
  [rd_go] -> read_gen/1(go)
  [proc_d256_0] -> Delay4/1
  [proc_sync] -> sync_generator/2(proc_sync)  "PROC_sync"
  [hmc_sync0] -> sync_generator/1(hmc_sync)  "HMC_sync"
  Delay4/1 -> [wr_d256_0]  "WR_d256"
  Delay7/1 -> [wr_en]  "WR_en"
  Delay12/1 -> [wr_addr]  "WR_addr"
  Delay16/1 -> [rd_bank]  "RD_bank"
  Delay15/1 -> [rd_go]  "RD_go"
  Delay14/1 -> [rd_en]  "RD_en"
  Delay13/1 -> [rd_mux_sel]  "RD_muxsel"
  Delay17/1 -> [rd_addr]  "RD_addr"
  Delay18/1 -> [rd_busy]  "RD_busy"
  sync_generator/1(sync) -> [rd_sync]  "RD_sync"
  [rd_sync] -> Delay6/1
  [ct_freq_gen_offset] -> gen_freq_calc/3(freq_offset)
  tag_reorder/5(out_err_missing0) -> [obuf_proc_err_miss_0_g]
  munge4/1(dout) -> [obuf0]
  dv1/1 -> Assert5/1  "IN_dv"
  tag1/1 -> Assert6/1
  din1/1 -> Assert7/1
  Assert5/1 -> [hmc_dv1]
  Assert6/1 -> [hmc_tag1]
  Assert7/1 -> [hmc_d2561]
  tag_reorder/4(do1) -> [proc_d256_1]
  tag_reorder/6(out_err_missing1) -> [obuf_proc_err_miss_1_g]
  [hmc_d2561] -> tag_reorder/7(d1)
  [hmc_tag1] -> tag_reorder/6(tag1)
  [hmc_dv1] -> tag_reorder/5(dv1)
  [proc_d256_1] -> Delay19/1
  Concat10/1 -> [dbuf7]
  Concat12/1 -> [dbuf6]
  Concat9/1 -> [dbuf5]
  Concat8/1 -> [dbuf4]
  Concat7/1 -> [dbuf3]
  Concat6/1 -> [dbuf2]
  Concat5/1 -> [dbuf1]
  Concat4/1 -> [dbuf0]
  [p0f7] -> Concat10/1
  [p0f6] -> Concat12/1
  [p1f5] -> Concat9/2
  [p0f5] -> Concat9/1
  [p1f4] -> Concat8/2
  [p0f4] -> Concat8/1
  [p1f3] -> Concat7/2
  [p0f3] -> Concat7/1
  [p1f2] -> Concat6/2
  [p0f2] -> Concat6/1
  [p0f1] -> Concat5/1
  [p1f1] -> Concat5/2
  [p1f7] -> Concat10/2
  [p1f6] -> Concat12/2
  [p1f0] -> Concat4/2
  [p0f0] -> Concat4/1
  bus_expand2/4(out13) -> [p0f3]  "d256_f3"
  bus_expand2/3(out14) -> [p0f2]  "d256_f2"
  bus_expand2/2(out15) -> [p0f1]  "d256_f1"
  bus_expand2/1(msb_out16) -> [p0f0]  "d256_f0"
  [wr_d256_0] -> bus_expand2/1(bus_in)
  Delay19/1 -> [wr_d256_1]
  [wr_d256_1] -> bus_expand4/1(bus_in)
  bus_expand4/1(msb_out16) -> [p1f0]
  bus_expand4/2(out15) -> [p1f1]
  bus_expand4/8(out9) -> [p1f7]
  bus_expand4/7(out10) -> [p1f6]
  bus_expand4/6(out11) -> [p1f5]
  bus_expand4/5(out12) -> [p1f4]
  bus_expand4/4(out13) -> [p1f3]
  bus_expand4/3(out14) -> [p1f2]
  bus_expand2/5(out12) -> [p0f4]
  bus_expand2/6(out11) -> [p0f5]
  bus_expand2/7(out10) -> [p0f6]
  bus_expand2/8(out9) -> [p0f7]
  bus_expand2/9(out8) -> [p0f8]  "d256_f4"
  bus_expand2/10(out7) -> [p0f9]  "d256_f5"
  bus_expand2/11(out6) -> [p0f10]  "d256_f6"
  bus_expand2/12(out5) -> [p0f11]  "d256_f7"
  bus_expand2/13(out4) -> [p0f12]
  bus_expand2/14(out3) -> [p0f13]
  bus_expand2/15(out2) -> [p0f14]
  bus_expand2/16(lsb_out1) -> [p0f15]
  bus_expand4/9(out8) -> [p1f8]
  bus_expand4/10(out7) -> [p1f9]
  bus_expand4/11(out6) -> [p1f10]
  bus_expand4/12(out5) -> [p1f11]
  bus_expand4/13(out4) -> [p1f12]
  bus_expand4/14(out3) -> [p1f13]
  bus_expand4/15(out2) -> [p1f14]
  bus_expand4/16(lsb_out1) -> [p1f15]
  Concat1/1 -> [dbuf15]
  Concat2/1 -> [dbuf14]
  Concat17/1 -> [dbuf13]
  Concat16/1 -> [dbuf12]
  Concat15/1 -> [dbuf11]
  Concat14/1 -> [dbuf10]
  Concat13/1 -> [dbuf9]
  Concat3/1 -> [dbuf8]
  [p0f15] -> Concat1/1
  [p0f14] -> Concat2/1
  [p1f13] -> Concat17/2
  [p0f13] -> Concat17/1
  [p1f12] -> Concat16/2
  [p0f12] -> Concat16/1
  [p1f11] -> Concat15/2
  [p0f11] -> Concat15/1
  [p1f10] -> Concat14/2
  [p0f10] -> Concat14/1
  [p0f9] -> Concat13/1
  [p1f9] -> Concat13/2
  [p1f15] -> Concat1/2
  [p1f14] -> Concat2/2
  [p1f8] -> Concat3/2
  [p0f8] -> Concat3/1
  [obuf10] -> pkt_data_mux/12
  [obuf8] -> pkt_data_mux/10
  [obuf9] -> pkt_data_mux/11
  [obuf14] -> pkt_data_mux/16
  [obuf12] -> pkt_data_mux/14
  [obuf15] -> pkt_data_mux/17
  [obuf13] -> pkt_data_mux/15
  [obuf11] -> pkt_data_mux/13
  [dbuf1] -> obuf1/2
  [wr_addr] -> obuf1/1
  [wr_en] -> obuf1/3
  [rd_addr] -> obuf1/4
  Constant1/1 -> obuf1/5
  Constant2/1 -> obuf1/6
  obuf1/2 -> munge1/1(din)
  obuf1/1 -> Terminator2/1
  munge1/1(dout) -> [obuf1]
  [dbuf2] -> obuf2/2
  [wr_addr] -> obuf2/1
  [wr_en] -> obuf2/3
  [rd_addr] -> obuf2/4
  Constant5/1 -> obuf2/5
  Constant6/1 -> obuf2/6
  obuf2/2 -> munge3/1(din)
  obuf2/1 -> Terminator10/1
  munge3/1(dout) -> [obuf2]
  [dbuf3] -> obuf3/2
  [wr_addr] -> obuf3/1
  [wr_en] -> obuf3/3
  [rd_addr] -> obuf3/4
  Constant3/1 -> obuf3/5
  Constant4/1 -> obuf3/6
  obuf3/2 -> munge2/1(din)
  obuf3/1 -> Terminator12/1
  munge2/1(dout) -> [obuf3]
  [dbuf4] -> obuf4/2
  [wr_addr] -> obuf4/1
  [wr_en] -> obuf4/3
  [rd_addr] -> obuf4/4
  Constant11/1 -> obuf4/5
  Constant12/1 -> obuf4/6
  obuf4/2 -> munge8/1(din)
  obuf4/1 -> Terminator14/1
  munge8/1(dout) -> [obuf4]
  [dbuf5] -> obuf5/2
  [wr_addr] -> obuf5/1
  [wr_en] -> obuf5/3
  [rd_addr] -> obuf5/4
  Constant7/1 -> obuf5/5
  Constant8/1 -> obuf5/6
  obuf5/2 -> munge5/1(din)
  obuf5/1 -> Terminator18/1
  munge5/1(dout) -> [obuf5]
  [dbuf6] -> obuf6/2
  [wr_addr] -> obuf6/1
  [wr_en] -> obuf6/3
  [rd_addr] -> obuf6/4
  Constant13/1 -> obuf6/5
  Constant14/1 -> obuf6/6
  obuf6/2 -> munge7/1(din)
  obuf6/1 -> Terminator13/1
  munge7/1(dout) -> [obuf6]
  [dbuf7] -> obuf7/2
  [wr_addr] -> obuf7/1
  [wr_en] -> obuf7/3
  [rd_addr] -> obuf7/4
  Constant9/1 -> obuf7/5
  Constant10/1 -> obuf7/6
  obuf7/2 -> munge6/1(din)
  obuf7/1 -> Terminator15/1
  munge6/1(dout) -> [obuf7]
  [dbuf8] -> obuf8/2
  [wr_addr] -> obuf8/1
  [wr_en] -> obuf8/3
  [rd_addr] -> obuf8/4
  Constant24/1 -> obuf8/5
  Constant25/1 -> obuf8/6
  obuf8/2 -> munge12/1(din)
  obuf8/1 -> Terminator20/1
  munge12/1(dout) -> [obuf8]
  [dbuf9] -> obuf9/2
  [wr_addr] -> obuf9/1
  [wr_en] -> obuf9/3
  [rd_addr] -> obuf9/4
  Constant15/1 -> obuf9/5
  Constant21/1 -> obuf9/6
  obuf9/2 -> munge9/1(din)
  obuf9/1 -> Terminator26/1
  munge9/1(dout) -> [obuf9]
  [dbuf10] -> obuf10/2
  [wr_addr] -> obuf10/1
  [wr_en] -> obuf10/3
  [rd_addr] -> obuf10/4
  Constant26/1 -> obuf10/5
  Constant27/1 -> obuf10/6
  obuf10/2 -> munge11/1(din)
  obuf10/1 -> Terminator19/1
  munge11/1(dout) -> [obuf10]
  [dbuf11] -> obuf11/2
  [wr_addr] -> obuf11/1
  [wr_en] -> obuf11/3
  [rd_addr] -> obuf11/4
  Constant22/1 -> obuf11/5
  Constant23/1 -> obuf11/6
  obuf11/2 -> munge10/1(din)
  obuf11/1 -> Terminator21/1
  munge10/1(dout) -> [obuf11]
  [dbuf12] -> obuf12/2
  [wr_addr] -> obuf12/1
  [wr_en] -> obuf12/3
  [rd_addr] -> obuf12/4
  Constant17/1 -> obuf12/5
  Constant18/1 -> obuf12/6
  obuf12/2 -> munge16/1(din)
  obuf12/1 -> Terminator23/1
  munge16/1(dout) -> [obuf12]
  [dbuf13] -> obuf13/2
  [wr_addr] -> obuf13/1
  [wr_en] -> obuf13/3
  [rd_addr] -> obuf13/4
  Constant28/1 -> obuf13/5
  Constant29/1 -> obuf13/6
  obuf13/2 -> munge13/1(din)
  obuf13/1 -> Terminator25/1
  munge13/1(dout) -> [obuf13]
  [dbuf14] -> obuf14/2
  [wr_addr] -> obuf14/1
  [wr_en] -> obuf14/3
  [rd_addr] -> obuf14/4
  Constant19/1 -> obuf14/5
  Constant20/1 -> obuf14/6
  obuf14/2 -> munge15/1(din)
  obuf14/1 -> Terminator22/1
  munge15/1(dout) -> [obuf14]
  [dbuf15] -> obuf15/2
  [wr_addr] -> obuf15/1
  [wr_en] -> obuf15/3
  [rd_addr] -> obuf15/4
  Constant30/1 -> obuf15/5
  Constant16/1 -> obuf15/6
  obuf15/2 -> munge14/1(din)
  obuf15/1 -> Terminator24/1
  munge14/1(dout) -> [obuf15]
  Gateway Out/1 -> Scope/1
  Gateway Out1/1 -> Scope/2
  Gateway Out2/1 -> Scope/3
  Gateway Out3/1 -> Scope/4
  Gateway Out4/1 -> Scope1/1
  Gateway Out5/1 -> Scope1/2
  Gateway Out6/1 -> Scope1/3
  Gateway Out7/1 -> Scope1/4
  [wr_addr] -> Gateway Out4/1
  [wr_en] -> Gateway Out5/1
  [rd_addr] -> Gateway Out6/1
  [rd_mux_sel] -> Gateway Out7/1
  Gateway Out8/1 -> Scope2/1
  Gateway Out9/1 -> Scope2/2
  Gateway Out10/1 -> Scope2/3
  Gateway Out11/1 -> Scope2/4
  [rd_addr] -> Gateway Out10/1
  [rd_mux_sel] -> Gateway Out11/1
  Gateway Out12/1 -> Scope3/1
  Gateway Out13/1 -> Scope3/2
  Gateway Out14/1 -> Scope3/3
  Gateway Out15/1 -> Scope3/4
  [rd_sync] -> Gateway Out12/1
  [rd_en] -> Gateway Out13/1
  [p0f0] -> Gateway Out14/1
  [p1f0] -> Gateway Out15/1
  Gateway Out18/1 -> Scope4/1
  Gateway Out19/1 -> Scope4/2
  Gateway Out16/1 -> Scope4/3
  Gateway Out17/1 -> Scope4/4
  Gateway Out20/1 -> Scope5/1
  Gateway Out21/1 -> Scope5/2
  Gateway Out22/1 -> Scope5/3
  Gateway Out23/1 -> Scope5/4
  [rd_sync] -> Gateway Out20/1
  [rd_en] -> Gateway Out21/1
  [p0f15] -> Gateway Out22/1
  [p1f15] -> Gateway Out23/1
  [rd_en] -> Gateway Out9/1
  [rd_sync] -> Gateway Out8/1
  Gateway Out30/1 -> Scope7/1
  Gateway Out31/1 -> Scope7/2
  Gateway Out28/1 -> Scope7/3
  Gateway Out29/1 -> Scope7/4
  [wr_addr] -> Gateway Out30/1
  [wr_en] -> Gateway Out31/1
  [dbuf0] -> Slice8/1, Slice7/1
  Gateway Out40/1 -> Scope10/1
  Gateway Out41/1 -> Scope10/2
  Gateway Out42/1 -> Scope10/3
  Gateway Out43/1 -> Scope10/4
  [wr_addr] -> Gateway Out40/1
  [proc_sync] -> Gateway Out41/1
  [rd_addr] -> Gateway Out42/1
  [rd_sync] -> Gateway Out43/1
  Slice7/1 -> Gateway Out28/1
  Slice8/1 -> Gateway Out29/1
  Gateway Out26/1 -> Scope6/1
  Gateway Out27/1 -> Scope6/2
  Gateway Out24/1 -> Scope6/3
  Gateway Out25/1 -> Scope6/4
  [rd_sync] -> Delay23/1
  [rd_en] -> Delay22/1
  Delay22/1 -> Gateway Out27/1
  Delay23/1 -> Gateway Out26/1
  [rd_addr] -> Delay24/1
  Delay24/1 -> Gateway Out24/1
  [obuf0] -> bus_expand/1(bus_in)
  Gateway Out33/1 -> Scope8/4
  Gateway Out34/1 -> Scope8/1
  Gateway Out35/1 -> Scope8/2
  Gateway Out32/1 -> Scope8/3
  Gateway Out38/1 -> Scope8/5
  Gateway Out36/1 -> Scope8/7
  Gateway Out37/1 -> Scope8/8
  Gateway Out39/1 -> Scope8/6
  bus_expand/1(msb_out8) -> Gateway Out34/1
  bus_expand/2(out7) -> Gateway Out35/1
  bus_expand/3(out6) -> Gateway Out32/1
  bus_expand/4(out5) -> Gateway Out33/1
  bus_expand/5(out4) -> Gateway Out38/1
  bus_expand/6(out3) -> Gateway Out39/1
  bus_expand/7(out2) -> Gateway Out36/1
  bus_expand/8(lsb_out1) -> Gateway Out37/1
  [obuf0] -> bus_expand1/1(bus_in)
  bus_expand1/1(msb_out8) -> Gateway Out25/1
  bus_expand1/2(out7) -> Gateway Out44/1
  bus_expand1/4(out5) -> Gateway Out45/1
  bus_expand1/6(out3) -> Gateway Out46/1
  bus_expand1/8(lsb_out1) -> Gateway Out47/1
  Gateway Out46/1 -> Scope6/7
  Gateway Out45/1 -> Scope6/6
  Gateway Out47/1 -> Scope6/8
  Gateway Out44/1 -> Scope6/5
  [wr_addr] -> Gateway Out18/1
  [dbuf15] -> Slice2/1
  [wr_en] -> Counter/2, Delay/2, Gateway Out16/1
  Delay/1 -> Relational/2
  Relational/1 -> Counter/1
  Counter/1 -> Gateway Out17/1
  Slice2/1 -> Relational/1, Delay/1, Gateway Out19/1

== system s_c_nbe_m32k/hmc_ct/pipeline ==
  d : Inport
  Register0 : xbsIndex_r4/Register  init=0  rst=off  en=off  dbl_ovrd=off  block_type=register
      settings: block_version=11.4
  Register1 : xbsIndex_r4/Register  init=0  rst=off  en=off  dbl_ovrd=off  block_type=register
      settings: block_version=11.4
  q : Outport
  wires:
  Register0/1 -> Register1/1
  d/1 -> Register0/1
  Register1/1 -> q/1

== system s_c_nbe_m32k/hmc_ct/pipeline1 ==
  d : Inport
  Register0 : xbsIndex_r4/Register  init=0  rst=off  en=off  dbl_ovrd=off  block_type=register
      settings: block_version=11.4
  Register1 : xbsIndex_r4/Register  init=0  rst=off  en=off  dbl_ovrd=off  block_type=register
      settings: block_version=11.4
  q : Outport
  wires:
  Register0/1 -> Register1/1
  d/1 -> Register0/1
  Register1/1 -> q/1

== system s_c_nbe_m32k/hmc_ct/pipeline10 ==
  d : Inport
  Register0 : xbsIndex_r4/Register  init=0  rst=off  en=off  dbl_ovrd=off  block_type=register
      settings: block_version=11.4
  Register1 : xbsIndex_r4/Register  init=0  rst=off  en=off  dbl_ovrd=off  block_type=register
      settings: block_version=11.4
  q : Outport
  wires:
  Register0/1 -> Register1/1
  d/1 -> Register0/1
  Register1/1 -> q/1
